simulink model "sim2"  (Simulink 8.1)
settings: Solver=ode45  StartTime=0.0  StopTime=10.0  RelTol=1e-3
settings Model: Creator=mohammad  LastModifiedBy=Mojtaba
settings DebuggingCC: FcnCallInpInsideContextMsg=EnableAllAsWarning
settings GRTTargetCC: CombineOutputUpdateFcns=on  GRTInterface=off

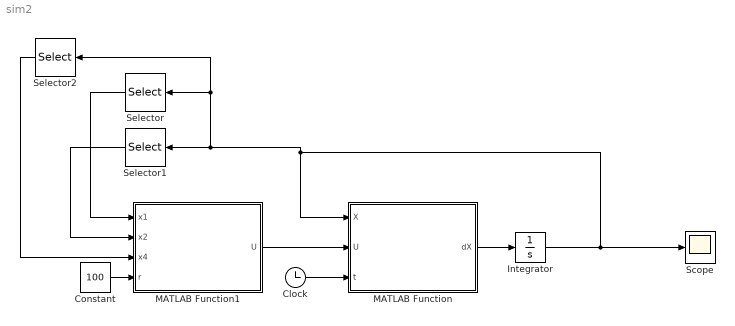
== system sim2 ==
  Clock : Clock
  Constant : Constant  Value=100
  Integrator : Integrator  InitialCondition=[0 0 0 0 0]
  MATLAB Function : MATLAB Function  TreatAsAtomicUnit=on
  MATLAB Function1 : MATLAB Function  TreatAsAtomicUnit=on
  Scope : Scope
  Selector : Selector  InputPortWidth=5  IndexOptions=Index vector (dialog)  Indices=[1]  OutputSizes=1
  Selector1 : Selector  InputPortWidth=5  IndexOptions=Index vector (dialog)  Indices=[2]  OutputSizes=1
  Selector2 : Selector  InputPortWidth=5  IndexOptions=Index vector (dialog)  Indices=[4]  OutputSizes=1
  wires:
  MATLAB Function/1(dX) -> Integrator/1
  Integrator/1 -> MATLAB Function/1(X), Selector1/1, Selector/1, Selector2/1, Scope/1
  MATLAB Function1/1(U) -> MATLAB Function/2(U)
  Clock/1 -> MATLAB Function/3(t)
  Selector/1 -> MATLAB Function1/1(x1)
  Selector1/1 -> MATLAB Function1/2(x2)
  Selector2/1 -> MATLAB Function1/3(x4)
  Constant/1 -> MATLAB Function1/4(r)

== matlab function MATLAB Function1 ==
  data: x1 input double; U output double; x2 input double; x4 input double; r input double
function U = fcn(x1,x2,x4,r)
%#codegen
Rs=1;
RM=0.005;
RA=0.001;
Rc=0.0398;
CR=4.4;
Cs=1.33;
CA=0.08;
Ls=0.0005;
Emax=2;
Emin=0.06;
Tmax=10; 
HR=1;
U=[(1/RM)*r;(1/RA)*r];

== matlab function MATLAB Function ==
  data: X input double; dX output double; U input double; t input double
function dX = fcn(X,U,t)
Rs=1;
RM=0.005;
RA=0.001;
Rc=0.0398;
CR=4.4;
Cs=1.33;
CA=0.08;
Ls=0.0005;
Emax=2;
Emin=0.06;
Tmax=10; 
HR=1;

tn=t/Tmax;
En=1.55*(((tn/0.7)^1.9)/((1+(tn/0.7)^1.9)))*(1/(1+(tn/1.17)^21.9));
E=(Emax-Emin)*En+Emin;
C=1/E;
dC=((589*(Emax - Emin)*((10*tn)/7)^(14/5))/(140*(((10*tn)/7)^(19/10) + 1)^2*(((100*tn)/117)^(219/10) + 1)) - (589*(Emax - Emin)*((10*tn)/7)^(9/10))/(140*(((10*tn)/7)^(19/10) + 1)*(((100*tn)/117)^(219/10) + 1)) + (2263*(Emax - Emin)*((10*tn)/7)^(19/10)*((100*tn)/117)^(209/10))/(78*(((10*tn)/7)^(19/10) + 1)*(((100*tn)/117)^(219/10) + 1)^2))/(Emin + (31*(Emax - Emin)*((10*tn)/7)^(19/10))/(20*(((10*tn)/7)^(19/10) + 1)*(((100*tn)/117)^(219/10) + 1)))^2;

A11=dC/C;
A22=-1/(Rs*CR);
A23=1/(Rs*CR);
A32=1/(Rs*Cs);
A33=-1/(Rs*Cs);
A35=1/Cs;
A45=-1/CA;
A53=-1/Ls;
A54=1/Ls;
A55=-Rc/Ls;
A=[A11 0 0 0 0;0 A22 A23 0 0;0 A32 A33 0 A35;0 0 0 0 A45;0 0 A53 A54 A55];

B11=1/C;
B12=-1/C;
B21=-1/CR;
B42=1/CA;
B=[B11 B12;B21 0;0 0;0 B42;0 0];

dX=A*X+B*U;
